simulink subsystem "Physics_Model"  (R2025b)
settings: Solver=VariableStepAuto  StartTime=0.0  StopTime=10.0  RelTol=1e-3
settings Model: Creator=Admin  LastModifiedBy=Admin

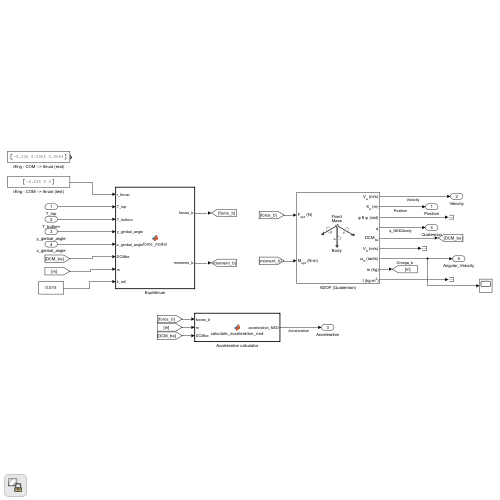
[thumbnail: Simulink's stored preview of the top-level diagram]
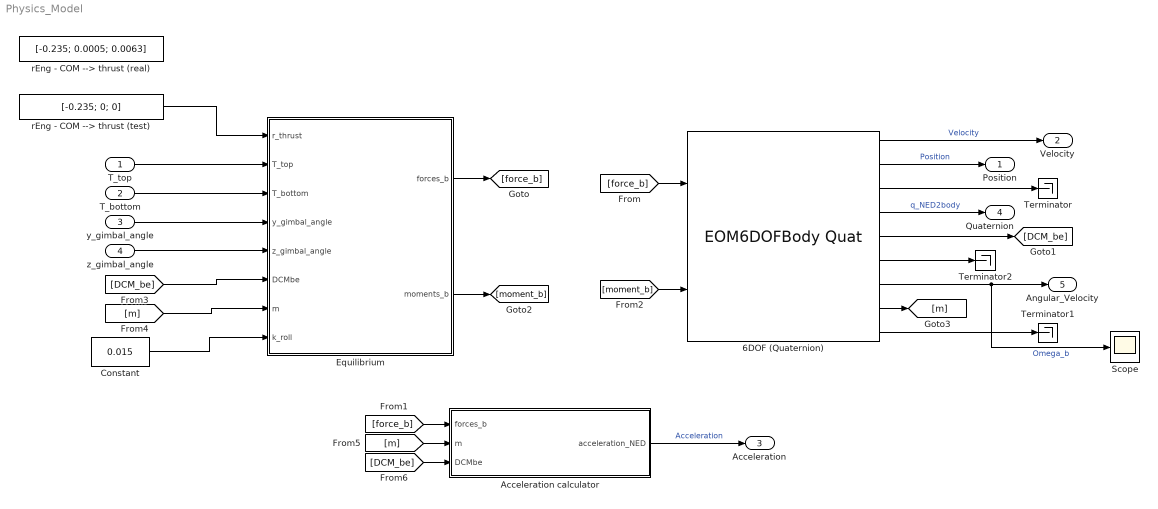
== system Physics_Model ==
  T_top : Inport
  T_bottom : Inport  Port=2
  y_gimbal_angle : Inport  Port=3
  z_gimbal_angle : Inport  Port=4
  6DOF (Quaternion) : EOM6DOFBodyQuat  eul_0=[0 pi/2 0]  mass_0=1.36  inertia=diag([7.5*10^-3, 0.08, 0.0831])  mass_flag=on
  Acceleration calculator : MATLAB Function  TreatAsAtomicUnit=on
  Constant : Constant  Value=0.015
  Equilibrium : MATLAB Function  TreatAsAtomicUnit=on
  Scope : Scope
      settings: ActiveDisplayYMinimum=-1  ActiveDisplayYMaximum=1  DataLoggingVariableName=ScopeData5
  Terminator : Terminator
  Terminator1 : Terminator
  Terminator2 : Terminator
  rEng - COM --> thrust (real) : Constant  Value=[-0.235; 0.0005; 0.0063]
  rEng - COM --> thrust (test) : Constant  Value=[-0.235; 0; 0]
  Position : Outport
  Velocity : Outport  Port=2
  Acceleration : Outport  Port=3
  Quaternion : Outport  Port=4
  Angular_Velocity : Outport  Port=5
  wires:
  6DOF (Quaternion)/6 -> Terminator2/1
  6DOF (Quaternion)/7 -> Angular_Velocity/1, Scope/1  "Omega_b"
  6DOF (Quaternion)/5 -> [DCM_be]
  [DCM_be] -> Acceleration calculator/3(DCMbe)
  Acceleration calculator/1(acceleration_NED) -> Acceleration/1  "Acceleration"
  6DOF (Quaternion)/9 -> Terminator1/1
  6DOF (Quaternion)/4 -> Quaternion/1  "q_NED2body"
  6DOF (Quaternion)/3 -> Terminator/1
  [m] -> Equilibrium/7(m)
  T_top/1 -> Equilibrium/2(T_top)
  6DOF (Quaternion)/1 -> Velocity/1  "Velocity"
  6DOF (Quaternion)/2 -> Position/1  "Position"
  [force_b] -> 6DOF (Quaternion)/1
  6DOF (Quaternion)/8 -> [m]
  [moment_b] -> 6DOF (Quaternion)/2
  T_bottom/1 -> Equilibrium/3(T_bottom)
  rEng - COM --> thrust (test)/1 -> Equilibrium/1(r_thrust)
  y_gimbal_angle/1 -> Equilibrium/4(y_gimbal_angle)
  z_gimbal_angle/1 -> Equilibrium/5(z_gimbal_angle)
  [DCM_be] -> Equilibrium/6(DCMbe)
  Constant/1 -> Equilibrium/8(k_roll)
  Equilibrium/1(forces_b) -> [force_b]
  Equilibrium/2(moments_b) -> [moment_b]
  [m] -> Acceleration calculator/2(m)
  [force_b] -> Acceleration calculator/1(forces_b)

== matlab function Physics_Model/Equilibrium ==
  data: r_thrust input; T_top input; T_bottom input; y_gimbal_angle input; z_gimbal_angle input; DCMbe input; m input; forces_b output; moments_b output; k_roll input
function [forces_b, moments_b] = force_model( ...
    r_thrust, T_top, T_bottom, ...
    y_gimbal_angle, z_gimbal_angle, ...
    DCMbe, m, k_roll)
%FORCE_MODEL Calculate total force and moment in body axes.
%
% Vehicle convention:
%   Nominal thrust axis = body +X
%   y_gimbal_angle produces body-Z thrust
%   z_gimbal_angle produces body-Y thrust
%
% DCMbe transforms NED -> body.
%
% Inputs:
%   r_thrust       [3x1] CoM to thrust point, body frame [m]
%   T_top          Top-propeller thrust [N]
%   T_bottom       Bottom-propeller thrust [N]
%   y_gimbal_angle Pitch-gimbal angle [rad]
%   z_gimbal_angle Yaw-gimbal angle [rad]
%   DCMbe          NED-to-body rotation matrix
%   m              Mass [kg]
%   k_roll         Differential-thrust roll coefficient
%
% Outputs:
%   forces_b       Total external force in body axes [N]
%   moments_b      Total moment about CoM in body axes [N*m]

T_total = T_top + T_bottom;
T_diff  = T_top - T_bottom;

%% Thrust direction

% This exactly reverses the controller definitions:
%
% pitch = atan2(Fz,Fx)
% yaw   = atan2(Fy,Fx)

thrust_direction_raw = [1;
                        tan(z_gimbal_angle);
                        tan(y_gimbal_angle)];

thrust_direction_b = ...
    thrust_direction_raw / norm(thrust_direction_raw);

T_b = T_total * thrust_direction_b;

%% Gravity

% NED +Z points downward
g = 9.81;
W_n = [0;0;m*g];

% DCMbe transforms NED -> body
W_b = DCMbe * W_n;

%% Total force

forces_b = T_b + W_b;

%% Moments

% Moment caused by applying thrust away from the CoM
M_tvc = cross(r_thrust, T_b);

% Roll moment generated by differential coaxial thrust
M_roll = [k_roll*T_diff;0;0];

moments_b = M_tvc + M_roll;

end

== matlab function Physics_Model/Acceleration calculator ==
  data: forces_b input; acceleration_NED output; m input; DCMbe input
function acceleration_NED = calculate_acceleration_ned( ...
    forces_b, m, DCMbe)
% Total inertial acceleration expressed in NED axes

acceleration_body = forces_b / m;
acceleration_NED = DCMbe.' * acceleration_body;

end
